simulink model "PVOutputSimulation2025a"  (R2025a)
settings: Solver=ode14x  StartTime=0  StopTime=(height(data)-1)*3600  FixedStep=3600  RelTol=1e-3
values from neighbouring files (symbols this model uses):
  temperaturePoints = temperaturePoints(:)    [generate_training_data_all_panels.m]
  vmpPoints = vmpPoints(:)    [generate_training_data_all_panels.m]
libraries: fl_lib x7, nesl_utility x5, ee_lib x1
settings Model: Creator=Asare  LastModifiedBy=Asare
settings SimscapeCC: SimscapeNominalValues="[{\"value\":\"1\",\"unit\":\"A\"},{\"value\":\"1\",\"unit\":\"bar\"},{\"value\":\"1\",\"unit\":\"cm^2\"},{\"value\":\"1\",\"unit\":\"cm^3/s\"},{\"value\":\"1\",\"unit\":\"kJ/kg\"},{\"value\":\"1\",\"unit\":\"kW\"},{\"value\":\"1\",\"unit\":\"l\"},{\"value\":\"1\",\"unit\":\"N\"},{\"value\":\"1\",\"unit\":\"N*m\"},{\"value\":\"1\",\"unit\":\"V\"},{\"value\":\"0.001\",\"unit\":\"Wb\"}]"  SimscapeLogType=all  SimscapeLogDataHistory=10000.0

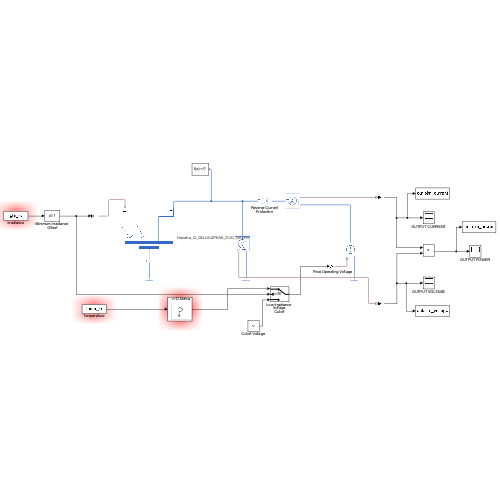
[thumbnail: Simulink's stored preview of the top-level diagram]
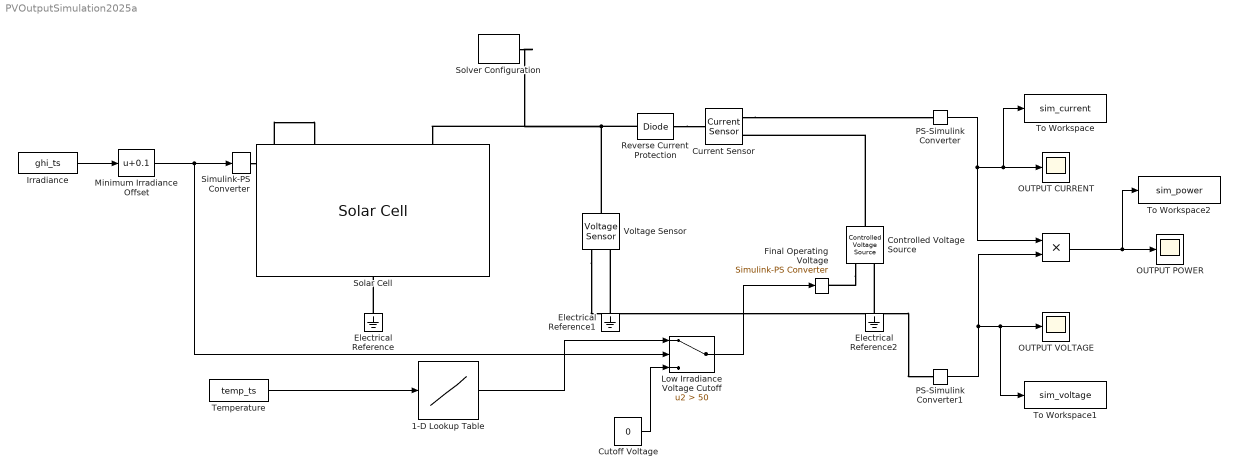
== system PVOutputSimulation2025a ==
  " " : Product
  1-D Lookup Table : Lookup_n-D  NumberOfTableDimensions=1  BreakpointsForDimension1=temperaturePoints  Table=vmpPoints  InterpMethod=Akima spline  InternalRulePriority=Speed  RndMeth=Simplest
  Controlled Voltage Source : fl_lib/Electrical/Electrical Sources/Controlled Voltage Source
  Current Sensor : fl_lib/Electrical/Electrical Sensors/Current Sensor
  Cutoff Voltage : Constant  Value=0
  Electrical Reference : fl_lib/Electrical/Electrical Elements/Electrical Reference
  Electrical Reference1 : fl_lib/Electrical/Electrical Elements/Electrical Reference
  Electrical Reference2 : fl_lib/Electrical/Electrical Elements/Electrical Reference
  Final Operating Voltage : nesl_utility/Simulink-PS Converter  PhysicalDomain=network_engine_domain  SubClassName=ps_input  LeftPortType=input  RightPortType=output  PseudoPeriodic=off  Frequencies=[]  NoiseDistribution=none  NoiseParameters=[]  Unit=V  AffineConversion=off  FilteringAndDerivatives=provide  SimscapeFilterOrder=1  InputFilterTimeConstant=0.001  UdotUserProvided=0
  Irradiance : FromWorkspace  VariableName=ghi_ts  SampleTime=3600
  Low Irradiance Voltage Cutoff : Switch  Criteria=u2 > Threshold  Threshold=50  SaturateOnIntegerOverflow=off  InputSameDT=off
  Minimum Irradiance Offset : Bias  Bias=0.1  SaturateOnIntegerOverflow=off
  OUTPUT CURRENT : Scope
      settings: ActiveDisplayYMinimum=-1.3233450719996423E-5  ActiveDisplayYMaximum=1.4642629839831067E-5
  OUTPUT POWER : Scope
      settings: ActiveDisplayYMinimum=-10336.969250763819  ActiveDisplayYMaximum=58349.956973621309
  OUTPUT VOLTAGE : Scope
      settings: ActiveDisplayYMinimum=-1092.4176124915666  ActiveDisplayYMaximum=703.79622288404107  DataLoggingVariableName=ScopeData2
  PS-Simulink Converter : nesl_utility/PS-Simulink Converter  PhysicalDomain=network_engine_domain  SubClassName=ps_output  LeftPortType=input  RightPortType=output  PseudoPeriodic=off  Frequencies=[]  VectorFormat=inherit  Unit=A  AffineConversion=off
  PS-Simulink Converter1 : nesl_utility/PS-Simulink Converter  PhysicalDomain=network_engine_domain  SubClassName=ps_output  LeftPortType=input  RightPortType=output  PseudoPeriodic=off  Frequencies=[]  VectorFormat=inherit  Unit=V  AffineConversion=off
  Reverse Current Protection : fl_lib/Electrical/Electrical Elements/Diode  Vf=0.6 V  Ron=0.001 Ohm  Goff=1e-8 1/Ohm  i_specify=off  i_priority=None  i=0 A  i_nominal_specify=off  i_nominal_value=1  i_nominal_unit=A  v_specify=off  v_priority=None  v=0 V  v_nominal_specify=off  v_nominal_value=1  v_nominal_unit=V
  Simulink-PS Converter : nesl_utility/Simulink-PS Converter  PhysicalDomain=network_engine_domain  SubClassName=ps_input  LeftPortType=input  RightPortType=output  PseudoPeriodic=off  Frequencies=[]  NoiseDistribution=none  NoiseParameters=[]  Unit=W/m^2  AffineConversion=off  FilteringAndDerivatives=provide  SimscapeFilterOrder=1  InputFilterTimeConstant=0.001  UdotUserProvided=0
  Solar Cell : ee_lib/Sources/Solar Cell  PartSpecification="{\"CollectionId\":\"SimscapeElectrical\",\"CollectionVersion\":\"1.0.0\",\"DatasetId\":\"Hanwha_Q_CELLS|QPEAK_DUO_G8_345|simscape.electrical.solarCell\",\"DisplayName\":\"Hanwha_Q_CELLS:QPEAK_DUO_G8_345\"}"  prm=3  Isc=5.3708 % Datasheet derived A  Voc=0.67543 % Datasheet derived V  Is=1.28579824698117e-07 % Datasheet derived A  Is2=5.34485351546167e-10 % Datasheet derived A  Iph=5.37077475429773 % Datasheet derived A  Ir0=1000 % Datasheet derived W/m^2  ec=1.49816908829742 % Datasheet derived  N2=1.33878321333864 % Datasheet derived  Rs=1.65840890236017e-06 % Datasheet derived Ohm  Rp=647.856546009085 % Datasheet derived Ohm  N_series=60 % Datasheet derived  N_parallel=2 % Datasheet derived  TIPH1=0.000254461499265197 % Datasheet derived 1/K  EG=1.12 % Datasheet derived eV  TXIS1=1.7025247110483 % Datasheet derived  TXIS2=21.8661940037091 % Datasheet derived  TRS1=0.238026082994793 % Datasheet derived  TRP1=0 % Parameter not set  Tmeas=25 % Datasheet derived degC  TFIXED=25 % Datasheet derived degC  thermal_mass=100 % Parameter not set J/K  initial_temperature=25 degC
      settings: AttributesFormatString=Hanwha_Q_CELLS:QPEAK_DUO_G8_345
  Solver Configuration : nesl_utility/Solver Configuration  PhysicalDomain=network_engine_domain  SubClassName=solver  LeftPortType=input  RightPortType=generic  Tones=[]  Harmonics=[]  SimulateNoise=off  Profile=off  UseLocalSampling=off  EnableSwitchedLinearOptims=on  FrequencyDomain=off  UseCCode=off  RelTol=0.001  AbsTol=0.001  MinStep=1e-09  ToWorkspace=off  RevertToSquareIcSolve=off  NumHomotopyIterations=100  PhasorMode=off  PhasorModeNumHarmonics=1  ConsistencySolver=NEWTON_XTOL_AFTER_FTOL  IndexReductionMethod=DerivativeReplacement  DoDC=off  ResidualTolerance=1e-09  ConsistencyTolSource=GLOBAL  ConsistencyAbsTol=0.001  ConsistencyRelTol=0.001  ConsistencyTolFactor=0.001  UseLocalSolver=off  LocalSolverChoice=NE_BACKWARD_EULER_ADVANCER  ResolveIndetEquations=on  FunctionEvalNumThread=1  LocalSolverSampleTime=3600  DoFixedCost=off  MaxNonlinIter=3  MaxModeIter=2  ComputeImpulses=off  ImpulseIterations=2  LinearAlgebra=auto  LinearAlgebraNumThread=0  EquationFormulation=NE_TIME_EF  DelaysMemoryBudget=1024  AutomaticFiltering=on  FilteringTimeConstant=0.001  PartitionStorageMethod=AS_NEEDED  PartitionMemoryBudget=1024  PartitionMethod=ROBUST  MultibodyUseLocalSolver=off  MultibodyLocalSolverChoice=ODE1  MultibodyLocalSolverSampleTime=0.001
  Temperature : FromWorkspace  VariableName=temp_ts  SampleTime=3600  OutputAfterFinalValue=Holding final value
  To Workspace : ToWorkspace  VariableName=sim_current  SampleTime=3600
  To Workspace1 : ToWorkspace  VariableName=sim_voltage  SampleTime=3600
  To Workspace2 : ToWorkspace  VariableName=sim_power  SampleTime=3600
  Voltage Sensor : fl_lib/Electrical/Electrical Sensors/Voltage Sensor
  wires:
  PS-Simulink Converter/1 -> " "/1, To Workspace/1, OUTPUT CURRENT/1
  PS-Simulink Converter1/1 -> " "/2, To Workspace1/1, OUTPUT VOLTAGE/1
  " "/1 -> To Workspace2/1, OUTPUT POWER/1
  Irradiance/1 -> Minimum Irradiance Offset/1
  Minimum Irradiance Offset/1 -> Low Irradiance Voltage Cutoff/2, Simulink-PS Converter/1
  Cutoff Voltage/1 -> Low Irradiance Voltage Cutoff/3
  Low Irradiance Voltage Cutoff/1 -> Final Operating Voltage/1
  Temperature/1 -> 1-D Lookup Table/1
  1-D Lookup Table/1 -> Low Irradiance Voltage Cutoff/1
  connections:
  Simulink-PS Converter/RConn1 -- Solar Cell/LConn1
  Electrical Reference/LConn1 -- Solar Cell/RConn1
  Electrical Reference1/LConn1 -- Voltage Sensor/RConn2
  Electrical Reference2/LConn1 -- Controlled Voltage Source/RConn2
  Controlled Voltage Source/LConn1 -- Current Sensor/RConn2
  Controlled Voltage Source/RConn1 -- Final Operating Voltage/RConn1
  Voltage Sensor/RConn1 -- PS-Simulink Converter1/LConn1
  Current Sensor/RConn1 -- PS-Simulink Converter/LConn1
  Reverse Current Protection/RConn1 -- Current Sensor/LConn1
  Reverse Current Protection/LConn1 -- Solver Configuration/RConn1 -- Solar Cell/LConn2 -- Voltage Sensor/LConn1
